simulink model "polarity_control"  (R2026a)
settings: Solver=FixedStepAuto  StopTime=inf  EnableMultiTasking=on
libraries: arduinolib x2, simulink x2
settings Model: SILPILModeSetting=veronly  ExtModeTrigDuration=2  Creator=cas_g  LastModifiedBy=00782620
settings HardwareCC: ProdBitPerInt=16.0  ProdBitPerPointer=16.0  ProdBitPerSizeT=16.0  ProdBitPerPtrDiffT=16.0  ProdWordSize=8.0  ProdHWDeviceType=Atmel->AVR
settings RTWCC: SystemTargetFile=ert.tlc  HardwareBoard=Arduino Uno  TLCOptions=-aInlineSetEventsForThisBaseRateFcn=TLC_FALSE -aSuppressMultiTaskScheduler=TLC_FALSE -aRateBasedStepFcn=1  Toolchain=Arduino AVR  BuildConfiguration=Faster Runs  Description=Embedded Coder
settings ERTTargetCC: ExtModeTransport=3.0  ExtModeAutomaticAllocSize=off  ExtModeStaticAllocSize=250.0  SupportContinuousTime=on  SupportVariableSizeSignals=on

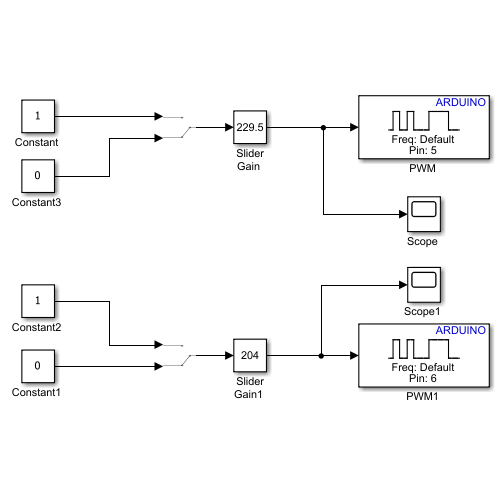
[thumbnail: Simulink's stored preview of the top-level diagram]
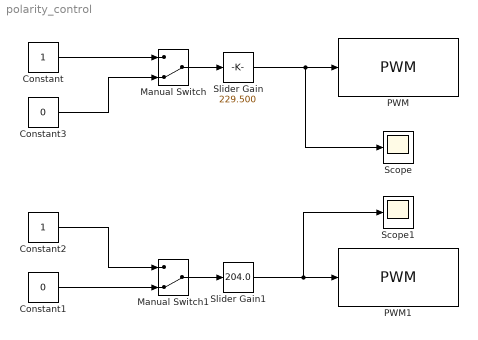
== system polarity_control ==
  "Constant " : Constant
  "Constant1 " : Constant  Value=0
  "Constant2 " : Constant
  "Constant3 " : Constant  Value=0
  Manual Switch : ManualSwitch  CurrentSetting=0
  Manual Switch1 : ManualSwitch  CurrentSetting=0
  "PWM " : arduinolib/PWM  pinNumber=5  frequencyType=Default  desiredFrequency=490.2  achievableFrequency=490.2
  "PWM1 " : arduinolib/PWM  pinNumber=6  frequencyType=Default  desiredFrequency=490.2  achievableFrequency=490.2
  "Scope " : Scope
      settings: ActiveDisplayYMinimum=-28.687499999999993  ActiveDisplayYMaximum=258.1875
  "Scope1 " : Scope
      settings: ActiveDisplayYMinimum=-31.874999999999993  ActiveDisplayYMaximum=286.875
  "Slider Gain " : simulink/Math Operations/Slider Gain  gain=229.500  low=0  high=255
  "Slider Gain1 " : simulink/Math Operations/Slider Gain  gain=204.0  low=0  high=255
  wires:
  Manual Switch/1 -> "Slider Gain "/1
  Manual Switch1/1 -> "Slider Gain1 "/1
  "Constant2 "/1 -> Manual Switch1/1
  "Constant1 "/1 -> Manual Switch1/2
  "Constant "/1 -> Manual Switch/1
  "Constant3 "/1 -> Manual Switch/2
  "Slider Gain "/1 -> "Scope "/1, "PWM "/1
  "Slider Gain1 "/1 -> "Scope1 "/1, "PWM1 "/1
